simulink model "ann_fresh_fault_scopes"  (R2024a)
settings: Solver=FixedStepDiscrete  StartTime=0.0  StopTime=0.26  FixedStep=5.0000000000000002e-05  RelTol=1e-3
InitFcn:
  | clear electrical_relay_live live_rms_features relay_block
undefined symbols (not defined in the file or in its folder): electrical_relay_live
libraries: spsRMSLib x8, spsThreePhasePISectionLineLib x2, spsThreePhaseFaultLib x1, spsThreePhaseParallelRLCLoadLib x1, spsThreePhaseVIMeasurementLib x1, spsThreePhaseSourceLib x1, spsThreePhaseTransformerTwoWindingsLib x1, spspowerguiLib x1
settings Model: Creator=crack  LastModifiedBy=crack

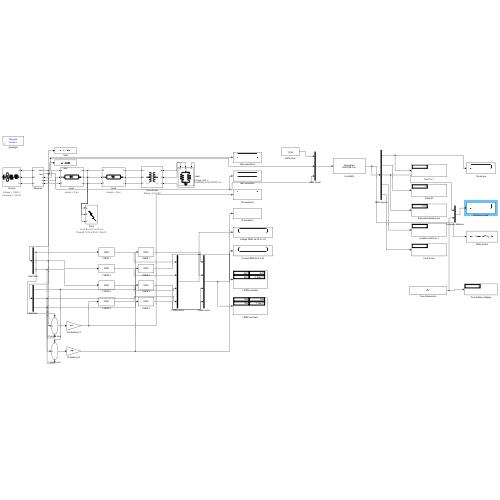
[thumbnail: Simulink's stored preview of the top-level diagram]
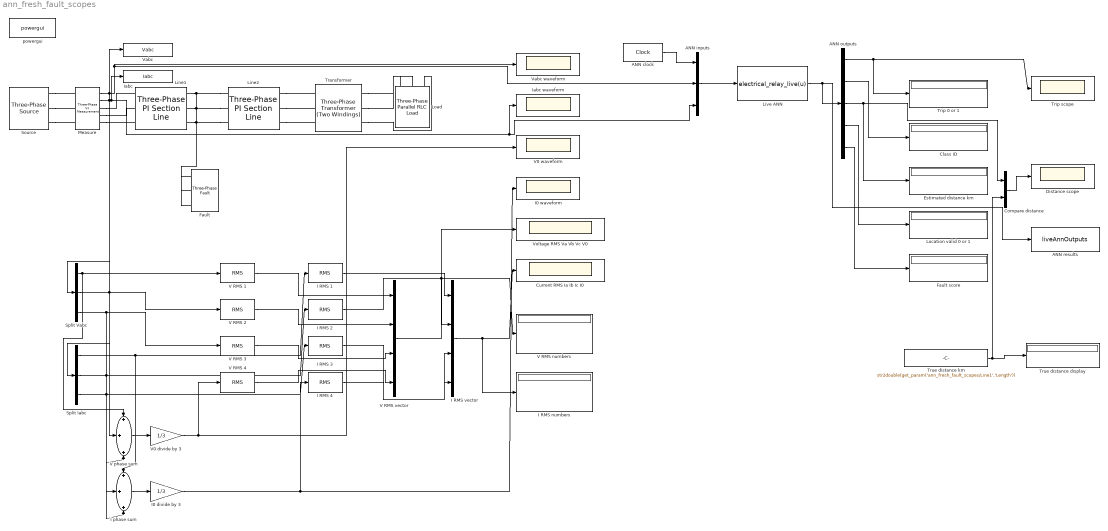
== system ann_fresh_fault_scopes ==
  ANN clock : DigitalClock  SampleTime=50e-6
  ANN inputs : Mux  Inputs=3
  ANN outputs : Demux  Outputs=5
  ANN results : ToWorkspace  VariableName=liveAnnOutputs  SaveFormat=Timeseries  SampleTime=-1
  Class ID : Display
  Compare distance : Mux  Inputs=2
  Current RMS Ia Ib Ic I0 : Scope
  Distance scope : Scope
  Estimated distance km : Display
  Fault : spsThreePhaseFaultLib/Three-Phase Fault  InitialStates=0  FaultA=on  FaultB=on  FaultC=on  GroundFault=on  SwitchTimes=[0.1 0.3]  External=off  SwitchStatus=NaN  FaultResistance=0.1  GroundResistance=0.1  SnubberResistance=1e6  SnubberCapacitance=inf  Measurements=None
      settings: AttributesFormatString=|
      | A=%<FaultA> B=%<FaultB> C=%<FaultC> G=%<GroundFault>
      | Time=%<SwitchTimes> s Rf=%<FaultResistance> Rg=%<GroundResistance>
  Fault score : Display
  I RMS {1..4} (4 alike) : spsRMSLib/RMS  TrueRMS=on  Freq=50  RMSInit=0  Ts=50e-6
  I RMS numbers : Display
  I RMS vector : Mux
  I phase sum : Sum  Inputs=+++
  I0 divide by 3 : Gain  Gain=1/3
  I0 waveform : Scope
  Iabc : ToWorkspace  VariableName=Iabc  SaveFormat=Timeseries  SampleTime=-1
  Iabc waveform : Scope
  Line1 : spsThreePhasePISectionLineLib/Three-Phase PI Section Line  LConnTagsString=a|b|c  RConnTagsString=A|B|C  Length=8  Frequency=50  Resistances=[0.01273 0.38640000000000002]  Inductances=[0.00093369999999999998 0.0041263999999999997]  Capacitances=[1.274e-08 7.7509999999999994e-09]
      settings: AttributesFormatString=Length = %<Length> km
  Line2 : spsThreePhasePISectionLineLib/Three-Phase PI Section Line  LConnTagsString=a|b|c  RConnTagsString=A|B|C  Length=3  Frequency=50  Resistances=[0.01273 0.38640000000000002]  Inductances=[0.00093369999999999998 0.0041263999999999997]  Capacitances=[1.274e-08 7.7509999999999994e-09]
      settings: AttributesFormatString=Length = %<Length> km
  Live ANN : MATLABFcn  MATLABFcn=electrical_relay_live(u)  OutputDimensions=5
  Load : spsThreePhaseParallelRLCLoadLib/Three-Phase Parallel RLC Load  LConnTagsString=A|B|C  Configuration=Y (grounded)  NominalVoltage=400  Vabc=[1e3 1e3 1e3]  Vabcp=[1e3 1e3 1e3]  NominalFrequency=50  UnbalancedPower=off  ActivePower=800000  InductivePower=300000  CapacitivePower=0  Pabc=[10e3 9e3 11e3]  QLabc=[100 90 110]  QCabc=[100 90 110]  Pabcp=[10e3 9e3 11e3]  QLabcp=[100 90 110]  QCabcp=[100 90 110]  Measurements=None  LoadType=constant Z
      settings: AttributesFormatString=|
      | Voltage=%<NominalVoltage> V
      | P=%<ActivePower> W Q=%<InductivePower> var
  Location valid 0 or 1 : Display
  Measure : spsThreePhaseVIMeasurementLib/Three-Phase V-I Measurement  VoltageMeasurement=phase-to-ground  SetLabelV=off  LabelV=Vabc  Vpu=off  VpuLL=off  CurrentMeasurement=yes  SetLabelI=off  LabelI=Iabc  Ipu=off  Pbase=100e6  Vbase=500e3  OutputType=Complex  PhasorSimulation=off  PSBequivalent=0
  Source : spsThreePhaseSourceLib/Three-Phase Source  InternalConnection=Yg  VoltagePhases=off  Voltage=11000  PhaseAngle=0  Voltage_phases=[25e3 25e3 25e3]/sqrt(3)  PhaseAngles_phases=[0 -120 +120]  Frequency=50  NonIdealSource=on  SpecifyImpedance=off  Resistance=4.0331316817904064  Inductance=0.00012837856865949445  ShortCircuitLevel=100e6  BaseVoltage=25e3  XRratio=7  BusType=swing  Pref=10e3  Qref=0  Prefabc=[10e3, 10e3, 10e3]  Qrefabc=[0, 0, 0]  Qmin=-inf  Qmax=inf
      settings: AttributesFormatString=|
      | Voltage = %<Voltage> V
      | Frequency = %<Frequency> Hz
  Split Iabc : Demux  Outputs=3
  Split Vabc : Demux  Outputs=3
  Transformer : spsThreePhaseTransformerTwoWindingsLib/Three-Phase Transformer (Two Windings)  Winding1Connection=Yg  Winding2Connection=Yg  CoreType=Three single-phase transformers  SetSaturation=off  Hysteresis=off  DataFile='hysteresis'  SetInitialFlux=off  Measurements=None  UNITS=pu  NominalPower=[1e6 50]  Winding1=[11000 0.005 0.025]  Winding2=[400 0.005 0.025]  Rm=500  Lm=500  L0=0.5  Saturation=[ 0,0 ; 0.0024,1.2 ; 1.0,1.52 ]  InitialFluxes=[ 0.8 , -0.8 , 0.7 ]  BreakLoop=off  DiscreteSolver=Trapezoidal iterative  DataType=off  TransfoNumber=1
      settings: AttributesFormatString=Rating = %<NominalPower>
  Trip 0 or 1 : Display
  Trip scope : Scope
  True distance display : Display
  True distance km : Constant  Value=str2double(get_param('ann_fresh_fault_scopes/Line1','Length'))
  V RMS {1..4} (4 alike) : spsRMSLib/RMS  TrueRMS=on  Freq=50  RMSInit=0  Ts=50e-6
  V RMS numbers : Display
  V RMS vector : Mux
  V phase sum : Sum  Inputs=+++
  V0 divide by 3 : Gain  Gain=1/3
  V0 waveform : Scope
  Vabc : ToWorkspace  VariableName=Vabc  SaveFormat=Timeseries  SampleTime=-1
  Vabc waveform : Scope
  Voltage RMS Va Vb Vc V0 : Scope
  powergui : spspowerguiLib/powergui  Priority=1  SimulationMode=Discrete  SampleTime=5.0000000000000002e-05  frequency=60  Iterations=50  frequencyindice=50  Pbase=100e6  ErrMax=1e-4  UnitsV=kV  UnitsW=MW  buscounter=0  FunctionMessages=off  echomessages=off  EnableUseOfTLC=off  CurrentSourceSwitches=off  DisableSnubberDevices=off  DisableRonSwitches=off  DisableVfSwitches=off  DisplayEquations=off  AutomaticDiscreteSolvers=off  SolverType=Tustin/Backward Euler (TBE)  Interpol=off  ExternalGateDelay=off  methode=off  Ts=100  x0status=blocks  SPID=on  SwTol=0  HookPort=off  NonlinearTolerance=1e-4  nMaxIteration=100  ContinueOnMaxIteration=off  RestoreLinks=warning  ResistiveCurrentMeasurement=off  Frange=[0:2:500]  Ylog=off  Xlog=on  ShowGrid=off  save=off  variable=ZData  structure=0  ZoomFFT=off  StartTime=0.0  cycles=1  DisplayStyle=1  fundamental=60  FreqAxis=off  MaxFrequency=1000  frequencyindicesteady=1  RmsSteady=1  display=off
  wires:
  Measure/1 -> Vabc waveform/1, ANN inputs/2, Vabc/1, Split Vabc/1
  Measure/2 -> Iabc waveform/1, ANN inputs/3, Iabc/1, Split Iabc/1
  Split Vabc/1 -> V phase sum/1, V RMS 1/1
  Split Iabc/1 -> I phase sum/1, I RMS 1/1
  Split Vabc/2 -> V phase sum/2, V RMS 2/1
  Split Iabc/2 -> I phase sum/2, I RMS 2/1
  Split Vabc/3 -> V phase sum/3, V RMS 3/1
  Split Iabc/3 -> I phase sum/3, I RMS 3/1
  V phase sum/1 -> V0 divide by 3/1
  I phase sum/1 -> I0 divide by 3/1
  V0 divide by 3/1 -> V0 waveform/1, V RMS 4/1
  I0 divide by 3/1 -> I0 waveform/1, I RMS 4/1
  V RMS 1/1 -> V RMS vector/1
  I RMS 1/1 -> I RMS vector/1
  V RMS 2/1 -> V RMS vector/2
  I RMS 2/1 -> I RMS vector/2
  V RMS 3/1 -> V RMS vector/3
  I RMS 3/1 -> I RMS vector/3
  V RMS 4/1 -> V RMS vector/4
  I RMS 4/1 -> I RMS vector/4
  V RMS vector/1 -> Voltage RMS Va Vb Vc V0/1, V RMS numbers/1
  I RMS vector/1 -> Current RMS Ia Ib Ic I0/1, I RMS numbers/1
  ANN clock/1 -> ANN inputs/1
  ANN inputs/1 -> Live ANN/1
  Live ANN/1 -> ANN outputs/1, ANN results/1
  ANN outputs/1 -> Trip 0 or 1/1, Trip scope/1
  ANN outputs/2 -> Class ID/1
  ANN outputs/3 -> Estimated distance km/1, Compare distance/1
  ANN outputs/4 -> Location valid 0 or 1/1
  ANN outputs/5 -> Fault score/1
  True distance km/1 -> True distance display/1, Compare distance/2
  Compare distance/1 -> Distance scope/1
  connections:
  Source/RConn1 -- Measure/LConn1
  Source/RConn2 -- Measure/LConn2
  Source/RConn3 -- Measure/LConn3
  Measure/RConn1 -- Line1/LConn1
  Measure/RConn2 -- Line1/LConn2
  Measure/RConn3 -- Line1/LConn3
  Line2/LConn1 -- Line1/RConn1 -- Fault/LConn1
  Line2/LConn2 -- Line1/RConn2 -- Fault/LConn2
  Line2/LConn3 -- Line1/RConn3 -- Fault/LConn3
  Line2/RConn1 -- Transformer/LConn1
  Line2/RConn2 -- Transformer/LConn2
  Line2/RConn3 -- Transformer/LConn3
  Transformer/RConn1 -- Load/LConn1
  Transformer/RConn2 -- Load/LConn2
  Transformer/RConn3 -- Load/LConn3
